simulink library "cylPackParChnlsLumped"  (R2025a)
settings: Solver=VariableStepAuto  StartTime=0.0  StopTime=10.0  RelTol=1e-3
undefined symbols (not defined in the file or in its folder): battery_builder_rtmsupport, gcbh
libraries: cylPackParChnlsLumped_lib x10, nesl_utility x3, batt_lib x1
(part 2 of 2)

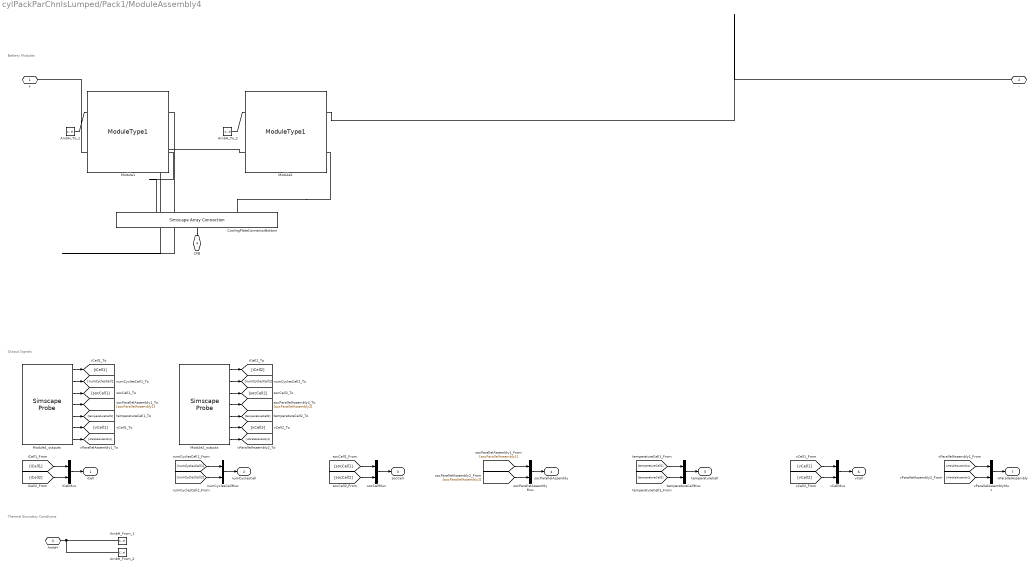
== system cylPackParChnlsLumped/Pack1/ModuleAssembly4 ==
  note: Thermal Boundary Conditions
  note: Output Signals
  note: Battery Modules
  AmbH_From_1 : ConnectionLabel  Label=ambH_1
  AmbH_From_2 : ConnectionLabel  Label=ambH_2
  AmbH_To_1 : ConnectionLabel  Label=ambH_1
  AmbH_To_2 : ConnectionLabel  Label=ambH_2
  CoolingPlateConnectorBottom : SimscapeArrayConnection  Domain=foundation.thermal.thermal  Mode=Sized Elements
  Module1 : cylPackParChnlsLumped_lib/Modules/ModuleType1  SOC_vecCell=ModuleType1.SOC_vecCell  T_vecCell=ModuleType1.T_vecCell K  V0_matCell=ModuleType1.V0_matCell V  V_rangeCell=ModuleType1.V_rangeCell V  R0_matCell=ModuleType1.R0_matCell Ohm  AHCell=ModuleType1.AHCell A*hr  extrapolation_optionCell=simscape.enum.extrapolation.nearest  thermal_massCell=ModuleType1.thermal_massCell J/K  CoolantResistance=ModuleType1.CoolantResistance K/W  AmbientResistance=ModuleType1.AmbientResistance K/W  P=32  S=12  iCell_specify=on  iCell_priority=None  iCell=ModuleAssembly4.Module1.iCell A  iCell_nominal_specify=off  iCell_nominal_value=1  iCell_nominal_unit=A  vCell_specify=on  vCell_priority=None  vCell=ModuleAssembly4.Module1.vCell V  vCell_nominal_specify=off  vCell_nominal_value=1  vCell_nominal_unit=V  socCell_specify=on  socCell_priority=High  socCell=ModuleAssembly4.Module1.socCell  socCell_nominal_specify=off  socCell_nominal_value=1  socCell_nominal_unit=1  numCyclesCell_specify=on  numCyclesCell_priority=High  numCyclesCell=ModuleAssembly4.Module1.numCyclesCell  numCyclesCell_nominal_specify=off  numCyclesCell_nominal_value=1  numCyclesCell_nominal_unit=1  temperatureCell_specify=on  temperatureCell_priority=High  temperatureCell=ModuleAssembly4.Module1.temperatureCell K  temperatureCell_nominal_specify=off  temperatureCell_nominal_value=1  temperatureCell_nominal_unit=K  vParallelAssembly_specify=on  vParallelAssembly_priority=None  vParallelAssembly=ModuleAssembly4.Module1.vParallelAssembly V  vParallelAssembly_nominal_specify=off  vParallelAssembly_nominal_value=1  vParallelAssembly_nominal_unit=V  socParallelAssembly_specify=on  socParallelAssembly_priority=None  socParallelAssembly=ModuleAssembly4.Module1.socParallelAssembly  socParallelAssembly_nominal_specify=off  socParallelAssembly_nominal_value=1  socParallelAssembly_nominal_unit=1
      settings: InternalSimscapePortConfiguration="{\"Bottom\":[{\"id\":\"n\",\"label\":\"-\",\"type\":\"foundation.electrical.electrical\"},{\"id\":\"BottomExtClnt\",\"label\":\"CPB\",\"type\":\"foundation.thermal.thermal\"}],\"Left\":[{\"id\":\"AmbH\",\"label\":\"AmbH\",\"type\":\"foundation.thermal.thermal\"}],\"Right\":[],\"Top\":[{\"id\":\"p\",\"label\":\"+\",\"type\":\"foundation.electrical.electrical\"}]}"
  Module1_outputs : SimscapeProbe  BoundBlock=245  Variables="{\"iCell\":{\"Probing\":\"ON\"},\"numCyclesCell\":{\"Probing\":\"ON\"},\"socCell\":{\"Probing\":\"ON\"},\"socParallelAssembly\":{\"Probing\":\"ON\"},\"temperatureCell\":{\"Probing\":\"ON\"},\"vCell\":{\"Probing\":\"ON\"},\"vParallelAssembly\":{\"Probing\":\"ON\"}}"
  Module2 : cylPackParChnlsLumped_lib/Modules/ModuleType1  SOC_vecCell=ModuleType1.SOC_vecCell  T_vecCell=ModuleType1.T_vecCell K  V0_matCell=ModuleType1.V0_matCell V  V_rangeCell=ModuleType1.V_rangeCell V  R0_matCell=ModuleType1.R0_matCell Ohm  AHCell=ModuleType1.AHCell A*hr  extrapolation_optionCell=simscape.enum.extrapolation.nearest  thermal_massCell=ModuleType1.thermal_massCell J/K  CoolantResistance=ModuleType1.CoolantResistance K/W  AmbientResistance=ModuleType1.AmbientResistance K/W  P=32  S=12  iCell_specify=on  iCell_priority=None  iCell=ModuleAssembly4.Module2.iCell A  iCell_nominal_specify=off  iCell_nominal_value=1  iCell_nominal_unit=A  vCell_specify=on  vCell_priority=None  vCell=ModuleAssembly4.Module2.vCell V  vCell_nominal_specify=off  vCell_nominal_value=1  vCell_nominal_unit=V  socCell_specify=on  socCell_priority=High  socCell=ModuleAssembly4.Module2.socCell  socCell_nominal_specify=off  socCell_nominal_value=1  socCell_nominal_unit=1  numCyclesCell_specify=on  numCyclesCell_priority=High  numCyclesCell=ModuleAssembly4.Module2.numCyclesCell  numCyclesCell_nominal_specify=off  numCyclesCell_nominal_value=1  numCyclesCell_nominal_unit=1  temperatureCell_specify=on  temperatureCell_priority=High  temperatureCell=ModuleAssembly4.Module2.temperatureCell K  temperatureCell_nominal_specify=off  temperatureCell_nominal_value=1  temperatureCell_nominal_unit=K  vParallelAssembly_specify=on  vParallelAssembly_priority=None  vParallelAssembly=ModuleAssembly4.Module2.vParallelAssembly V  vParallelAssembly_nominal_specify=off  vParallelAssembly_nominal_value=1  vParallelAssembly_nominal_unit=V  socParallelAssembly_specify=on  socParallelAssembly_priority=None  socParallelAssembly=ModuleAssembly4.Module2.socParallelAssembly  socParallelAssembly_nominal_specify=off  socParallelAssembly_nominal_value=1  socParallelAssembly_nominal_unit=1
      settings: InternalSimscapePortConfiguration="{\"Bottom\":[{\"id\":\"n\",\"label\":\"-\",\"type\":\"foundation.electrical.electrical\"},{\"id\":\"BottomExtClnt\",\"label\":\"CPB\",\"type\":\"foundation.thermal.thermal\"}],\"Left\":[{\"id\":\"AmbH\",\"label\":\"AmbH\",\"type\":\"foundation.thermal.thermal\"}],\"Right\":[],\"Top\":[{\"id\":\"p\",\"label\":\"+\",\"type\":\"foundation.electrical.electrical\"}]}"
  Module2_outputs : SimscapeProbe  BoundBlock=247  Variables="{\"iCell\":{\"Probing\":\"ON\"},\"numCyclesCell\":{\"Probing\":\"ON\"},\"socCell\":{\"Probing\":\"ON\"},\"socParallelAssembly\":{\"Probing\":\"ON\"},\"temperatureCell\":{\"Probing\":\"ON\"},\"vCell\":{\"Probing\":\"ON\"},\"vParallelAssembly\":{\"Probing\":\"ON\"}}"
  iCellMux : Mux  Inputs=2
  numCyclesCellMux : Mux  Inputs=2
  socCellMux : Mux  Inputs=2
  socParallelAssemblyMux : Mux  Inputs=2
  temperatureCellMux : Mux  Inputs=2
  vCellMux : Mux  Inputs=2
  vParallelAssemblyMux : Mux  Inputs=2
  + : PMIOPort  Side=Left
  - : PMIOPort  Port=2  Side=Right
  AmbH : PMIOPort  Port=3  Side=Right  ConnectionType=Connection: foundation.thermal.thermal
  CPB : PMIOPort  Port=4  Side=Right  ConnectionType=Connection: foundation.thermal.thermal
  iCell : Outport
  numCyclesCell : Outport  Port=2
  socCell : Outport  Port=3
  socParallelAssembly : Outport  Port=4
  temperatureCell : Outport  Port=5
  vCell : Outport  Port=6
  vParallelAssembly : Outport  Port=7
  wires:
  [vParallelAssembly2] -> vParallelAssemblyMux/2
  Module2_outputs/7 -> [vParallelAssembly2]
  [vCell2] -> vCellMux/2
  Module2_outputs/6 -> [vCell2]
  [temperatureCell2] -> temperatureCellMux/2
  Module2_outputs/5 -> [temperatureCell2]
  [socParallelAssembly2] -> socParallelAssemblyMux/2
  Module2_outputs/4 -> [socParallelAssembly2]
  [socCell2] -> socCellMux/2
  Module2_outputs/3 -> [socCell2]
  [numCyclesCell2] -> numCyclesCellMux/2
  Module2_outputs/2 -> [numCyclesCell2]
  [iCell2] -> iCellMux/2
  Module2_outputs/1 -> [iCell2]
  [vParallelAssembly1] -> vParallelAssemblyMux/1
  vParallelAssemblyMux/1 -> vParallelAssembly/1
  Module1_outputs/7 -> [vParallelAssembly1]
  [vCell1] -> vCellMux/1
  vCellMux/1 -> vCell/1
  Module1_outputs/6 -> [vCell1]
  [temperatureCell1] -> temperatureCellMux/1
  temperatureCellMux/1 -> temperatureCell/1
  Module1_outputs/5 -> [temperatureCell1]
  [socParallelAssembly1] -> socParallelAssemblyMux/1
  socParallelAssemblyMux/1 -> socParallelAssembly/1
  Module1_outputs/4 -> [socParallelAssembly1]
  [socCell1] -> socCellMux/1
  socCellMux/1 -> socCell/1
  Module1_outputs/3 -> [socCell1]
  [numCyclesCell1] -> numCyclesCellMux/1
  numCyclesCellMux/1 -> numCyclesCell/1
  Module1_outputs/2 -> [numCyclesCell1]
  [iCell1] -> iCellMux/1
  iCellMux/1 -> iCell/1
  Module1_outputs/1 -> [iCell1]
  connections:
  CoolingPlateConnectorBottom/RConn1 -- CPB/RConn1
  CoolingPlateConnectorBottom/LConn2 -- Module2/RConn2
  CoolingPlateConnectorBottom/LConn1 -- Module1/RConn2
  AmbH_To_2/LConn1 -- Module2/LConn1
  AmbH_From_2/LConn1 -- AmbH_From_1/LConn1 -- AmbH/RConn1
  AmbH_To_1/LConn1 -- Module1/LConn1
  Module2/RConn1 -- -/RConn1
  Module1/LConn2 -- +/RConn1
  Module2/LConn2 -- Module1/RConn1
